simulink model "ModelCLLCController"  (R2026a)
settings: Solver=ode23t  StopTime=5e-3  FixedStep=1e-4  MaxStep=1e-6  AbsTol=1e-3
PreLoadFcn:
  | % Parameterize the model
  | 
  | if ~exist('CLLCDesign', 'var')
  | CLLCConverterDefaultInputParameters;
  | end
undefined symbols (not defined in the file or in its folder): CLLCController
libraries: fl_lib x46, nesl_utility x45, ee_lib x35, ConverterLibrary x1
(part 2 of 4)

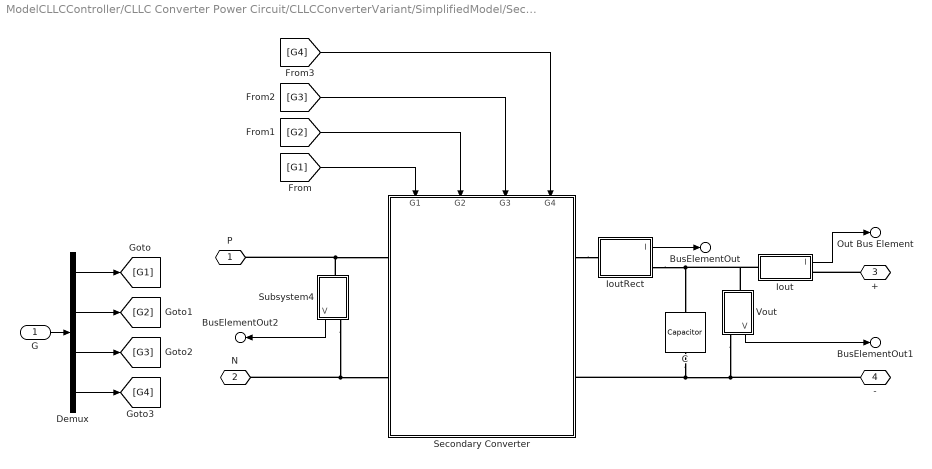
== system ModelCLLCController/CLLC Converter Power Circuit/CLLCConverterVariant/SimplifiedModel/Secondary Converter ==
  G : Inport
  C : fl_lib/Electrical/Electrical Elements/Capacitor  c=Co F  r=Rco Ohm  g=0 1/Ohm  i_specify=off  i_priority=None  i=0 A  i_nominal_specify=off  i_nominal_value=1  i_nominal_unit=A  v_specify=off  v_priority=None  v=450 V  v_nominal_specify=off  v_nominal_value=1  v_nominal_unit=V  vc_specify=on  vc_priority=High  vc=Vco V  vc_nominal_specify=off  vc_nominal_value=1  vc_nominal_unit=V
  Demux : Demux
  Iout : Subsystem
      mask Display: disp("I")
  IoutRect : Subsystem
      mask Display: disp("I")
  Secondary Converter : Subsystem  VariantControl=IdealSwitch
      settings: PortSchema="{\"entries\":[{\"content\":{\"sides\":[{\"content\":{\"connectorIds\":[\"LConn1\",\"LConn2\"]},\"type\":\"ConnectorPlacement.EquallySpacedRectSide\",\"uuid\":\"27c41940-d662-4779-afdd-48b642f77411\"},{\"content\":{\"connectorIds\":[\"RConn1\",\"RConn2\"],\"side\":\"RIGHT\"},\"type\":\"ConnectorPlacement.EquallySpacedRectSide\",\"uuid\":\"b0072b01-add1-4b0f-b94e-e1b6c9886b0e\"},{\"content\":{\"connectorIds\":[\"In1\",\"In2\",\"In3\",\"In4\"],\"side\":\"TOP\"},\"type\":\"ConnectorPlacement.EquallySpacedRectSide\",\"uuid\":\"c43bed80-422d-49db-9596-8b38d5c3e411\"},{\"content\":{\"side\":\"BOTTOM\"},\"type\":\"ConnectorPlacement.EquallySpacedRectSide\",\"uuid\":\"01f06046-f57e-45b0-bca5-368a5a543f97\"}]},\"type\":\"ConnectorPlacement.EquallySpacedConnector\",\"uuid\":\"2fcb5370-6bd7-4702-bf87-ebedbb7e376c\"}],\"packageUris\":[\"http://schema.mathworks.com/mf0/Connector/R2020b\"],\"version\":\"1.0\"}"
  Subsystem4 : Subsystem
      settings: PortSchema="{\"entries\":[{\"content\":{\"sides\":[{\"content\":{\"connectorIds\":[\"LConn1\"]},\"type\":\"ConnectorPlacement.EquallySpacedRectSide\",\"uuid\":\"e749c2ff-fd60-426f-a769-b61a7dfe80d2\"},{\"content\":{\"connectorIds\":[\"RConn1\",\"Out1\"],\"side\":\"RIGHT\"},\"type\":\"ConnectorPlacement.EquallySpacedRectSide\",\"uuid\":\"f3bb02bd-f8d2-4326-b68c-6f969fa4ac22\"},{\"content\":{\"side\":\"TOP\"},\"type\":\"ConnectorPlacement.EquallySpacedRectSide\",\"uuid\":\"9ab7a0d1-20d8-49e4-8eb3-54d34434204c\"}]},\"type\":\"ConnectorPlacement.EquallySpacedConnector\",\"uuid\":\"19e2a6d5-13f4-47de-bb59-b826817cba83\"}],\"packageUris\":[\"http://schema.mathworks.com/mf0/Connector/R2020b\"],\"version\":\"1.0\"}"
      mask Display: disp("V")
  Vout : Subsystem
      settings: PortSchema="{\"entries\":[{\"content\":{\"sides\":[{\"content\":{\"connectorIds\":[\"LConn1\"]},\"type\":\"ConnectorPlacement.EquallySpacedRectSide\",\"uuid\":\"e749c2ff-fd60-426f-a769-b61a7dfe80d2\"},{\"content\":{\"connectorIds\":[\"RConn1\",\"Out1\"],\"side\":\"RIGHT\"},\"type\":\"ConnectorPlacement.EquallySpacedRectSide\",\"uuid\":\"f3bb02bd-f8d2-4326-b68c-6f969fa4ac22\"},{\"content\":{\"side\":\"TOP\"},\"type\":\"ConnectorPlacement.EquallySpacedRectSide\",\"uuid\":\"9ab7a0d1-20d8-49e4-8eb3-54d34434204c\"}]},\"type\":\"ConnectorPlacement.EquallySpacedConnector\",\"uuid\":\"19e2a6d5-13f4-47de-bb59-b826817cba83\"}],\"packageUris\":[\"http://schema.mathworks.com/mf0/Connector/R2020b\"],\"version\":\"1.0\"}"
      mask Display: disp("V")
  P : PMIOPort  Side=Left
  N : PMIOPort  Port=2  Side=Left
  + : PMIOPort  Port=3  Side=Right
  - : PMIOPort  Port=4  Side=Right
  Out Bus Element : Outport  PortName=meas  Element=Iout [A]
  BusElementOut : Outport  PortName=meas  Element=IL [A]
  BusElementOut1 : Outport  PortName=meas  Element=Vout [V]
  BusElementOut2 : Outport  PortName=meas  Element=Vac [V]
  wires:
  Iout/1(I) -> Out Bus Element/1
  IoutRect/1(I) -> BusElementOut/1
  Vout/1(V) -> BusElementOut1/1
  Subsystem4/1(V) -> BusElementOut2/1
  Demux/2 -> [G2]
  Demux/1 -> [G1]
  G/1 -> Demux/1
  Demux/4 -> [G4]
  Demux/3 -> [G3]
  [G2] -> Secondary Converter/2(G2)
  [G3] -> Secondary Converter/3(G3)
  [G1] -> Secondary Converter/1(G1)
  [G4] -> Secondary Converter/4(G4)
  connections:
  Secondary Converter/RConn1 -- IoutRect/LConn1
  Subsystem4/RConn1 -- N/RConn1 -- Secondary Converter/LConn2
  Subsystem4/LConn1 -- P/RConn1 -- Secondary Converter/LConn1
  C/RConn1 -- -/RConn1 -- Vout/RConn1 -- Secondary Converter/RConn2
  IoutRect/RConn1 -- Iout/LConn1 -- Vout/LConn1 -- C/LConn1
  +/RConn1 -- Iout/RConn1

== system ModelCLLCController/CLLC Converter Power Circuit/CLLCConverterVariant/DetailedModel/Primary Converter/Iin ==
  Current Sensor : fl_lib/Electrical/Electrical Sensors/Current Sensor
  PS-Simulink Converter : nesl_utility/PS-Simulink Converter  PhysicalDomain=network_engine_domain  SubClassName=ps_output  LeftPortType=input  RightPortType=output  PseudoPeriodic=off  Frequencies=[]  VectorFormat=inherit  Unit=inherit  AffineConversion=off
  + : PMIOPort  Side=Left
  - : PMIOPort  Port=2  Side=Right
  I : Outport
  wires:
  PS-Simulink Converter/1 -> I/1
  connections:
  Current Sensor/RConn2 -- -/RConn1
  +/RConn1 -- Current Sensor/LConn1
  Current Sensor/RConn1 -- PS-Simulink Converter/LConn1

== system ModelCLLCController/CLLC Converter Power Circuit/CLLCConverterVariant/DetailedModel/Primary Converter/Primary Converter Full Bridge ==
  G1 : Inport
  G2 : Inport  Port=2
  G3 : Inport  Port=3
  G4 : Inport  Port=4
  Ideal MOSFET with Thermal : Subsystem  VariantControl=IdealMOSFETwithThermal
      settings: PortSchema="{\"entries\":[{\"content\":{\"sides\":[{\"content\":{\"connectorIds\":[\"LConn1\",\"LConn2\"]},\"type\":\"ConnectorPlacement.EquallySpacedRectSide\",\"uuid\":\"27c41940-d662-4779-afdd-48b642f77411\"},{\"content\":{\"connectorIds\":[\"RConn1\",\"RConn2\"],\"side\":\"RIGHT\"},\"type\":\"ConnectorPlacement.EquallySpacedRectSide\",\"uuid\":\"b0072b01-add1-4b0f-b94e-e1b6c9886b0e\"},{\"content\":{\"connectorIds\":[\"In1\",\"In2\",\"In3\",\"In4\"],\"side\":\"TOP\"},\"type\":\"ConnectorPlacement.EquallySpacedRectSide\",\"uuid\":\"c43bed80-422d-49db-9596-8b38d5c3e411\"},{\"content\":{\"side\":\"BOTTOM\"},\"type\":\"ConnectorPlacement.EquallySpacedRectSide\",\"uuid\":\"01f06046-f57e-45b0-bca5-368a5a543f97\"}]},\"type\":\"ConnectorPlacement.EquallySpacedConnector\",\"uuid\":\"2fcb5370-6bd7-4702-bf87-ebedbb7e376c\"}],\"packageUris\":[\"http://schema.mathworks.com/mf0/Connector/R2020b\"],\"version\":\"1.0\"}"
  Ideal Switch : Subsystem  VariantControl=IdealSwitch
      settings: PortSchema="{\"entries\":[{\"content\":{\"sides\":[{\"content\":{\"connectorIds\":[\"LConn1\",\"LConn2\"]},\"type\":\"ConnectorPlacement.EquallySpacedRectSide\",\"uuid\":\"27c41940-d662-4779-afdd-48b642f77411\"},{\"content\":{\"connectorIds\":[\"RConn1\",\"RConn2\"],\"side\":\"RIGHT\"},\"type\":\"ConnectorPlacement.EquallySpacedRectSide\",\"uuid\":\"b0072b01-add1-4b0f-b94e-e1b6c9886b0e\"},{\"content\":{\"connectorIds\":[\"In1\",\"In2\",\"In3\",\"In4\"],\"side\":\"TOP\"},\"type\":\"ConnectorPlacement.EquallySpacedRectSide\",\"uuid\":\"c43bed80-422d-49db-9596-8b38d5c3e411\"},{\"content\":{\"side\":\"BOTTOM\"},\"type\":\"ConnectorPlacement.EquallySpacedRectSide\",\"uuid\":\"01f06046-f57e-45b0-bca5-368a5a543f97\"}]},\"type\":\"ConnectorPlacement.EquallySpacedConnector\",\"uuid\":\"2fcb5370-6bd7-4702-bf87-ebedbb7e376c\"}],\"packageUris\":[\"http://schema.mathworks.com/mf0/Connector/R2020b\"],\"version\":\"1.0\"}"
  P1 : PMIOPort  Side=Left
  N1 : PMIOPort  Port=2  Side=Left
  P2 : PMIOPort  Port=3  Side=Right
  N2 : PMIOPort  Port=4  Side=Right

== system ModelCLLCController/CLLC Converter Power Circuit/CLLCConverterVariant/DetailedModel/Primary Converter/Vin ==
  PS-Simulink Converter : nesl_utility/PS-Simulink Converter  PhysicalDomain=network_engine_domain  SubClassName=ps_output  LeftPortType=input  RightPortType=output  PseudoPeriodic=off  Frequencies=[]  VectorFormat=inherit  Unit=inherit  AffineConversion=off
  Voltage Sensor : fl_lib/Electrical/Electrical Sensors/Voltage Sensor
  + : PMIOPort  Side=Left
  - : PMIOPort  Port=2  Side=Right
  V : Outport
  wires:
  PS-Simulink Converter/1 -> V/1
  connections:
  Voltage Sensor/RConn2 -- -/RConn1
  Voltage Sensor/LConn1 -- +/RConn1
  PS-Simulink Converter/LConn1 -- Voltage Sensor/RConn1

== system ModelCLLCController/CLLC Converter Power Circuit/CLLCConverterVariant/DetailedModel/Resonant Tank/Ip ==
  Current Sensor : fl_lib/Electrical/Electrical Sensors/Current Sensor
  PS-Simulink Converter : nesl_utility/PS-Simulink Converter  PhysicalDomain=network_engine_domain  SubClassName=ps_output  LeftPortType=input  RightPortType=output  PseudoPeriodic=off  Frequencies=[]  VectorFormat=inherit  Unit=inherit  AffineConversion=off
  + : PMIOPort  Side=Left
  - : PMIOPort  Port=2  Side=Right
  I : Outport
  wires:
  PS-Simulink Converter/1 -> I/1
  connections:
  Current Sensor/RConn2 -- -/RConn1
  +/RConn1 -- Current Sensor/LConn1
  Current Sensor/RConn1 -- PS-Simulink Converter/LConn1

== system ModelCLLCController/CLLC Converter Power Circuit/CLLCConverterVariant/DetailedModel/Resonant Tank/Is ==
  Current Sensor : fl_lib/Electrical/Electrical Sensors/Current Sensor
  PS-Simulink Converter : nesl_utility/PS-Simulink Converter  PhysicalDomain=network_engine_domain  SubClassName=ps_output  LeftPortType=input  RightPortType=output  PseudoPeriodic=off  Frequencies=[]  VectorFormat=inherit  Unit=inherit  AffineConversion=off
  + : PMIOPort  Side=Left
  - : PMIOPort  Port=2  Side=Right
  I : Outport
  wires:
  PS-Simulink Converter/1 -> I/1
  connections:
  Current Sensor/RConn2 -- -/RConn1
  +/RConn1 -- Current Sensor/LConn1
  Current Sensor/RConn1 -- PS-Simulink Converter/LConn1

== system ModelCLLCController/CLLC Converter Power Circuit/CLLCConverterVariant/DetailedModel/Resonant Tank/Vp ==
  PS-Simulink Converter : nesl_utility/PS-Simulink Converter  PhysicalDomain=network_engine_domain  SubClassName=ps_output  LeftPortType=input  RightPortType=output  PseudoPeriodic=off  Frequencies=[]  VectorFormat=inherit  Unit=inherit  AffineConversion=off
  Voltage Sensor : fl_lib/Electrical/Electrical Sensors/Voltage Sensor
  + : PMIOPort  Side=Left
  - : PMIOPort  Port=2  Side=Right
  V : Outport
  wires:
  PS-Simulink Converter/1 -> V/1
  connections:
  Voltage Sensor/RConn2 -- -/RConn1
  Voltage Sensor/LConn1 -- +/RConn1
  PS-Simulink Converter/LConn1 -- Voltage Sensor/RConn1

== system ModelCLLCController/CLLC Converter Power Circuit/CLLCConverterVariant/DetailedModel/Resonant Tank/Vs ==
  PS-Simulink Converter : nesl_utility/PS-Simulink Converter  PhysicalDomain=network_engine_domain  SubClassName=ps_output  LeftPortType=input  RightPortType=output  PseudoPeriodic=off  Frequencies=[]  VectorFormat=inherit  Unit=inherit  AffineConversion=off
  Voltage Sensor : fl_lib/Electrical/Electrical Sensors/Voltage Sensor
  + : PMIOPort  Side=Left
  - : PMIOPort  Port=2  Side=Right
  V : Outport
  wires:
  PS-Simulink Converter/1 -> V/1
  connections:
  Voltage Sensor/RConn2 -- -/RConn1
  Voltage Sensor/LConn1 -- +/RConn1
  PS-Simulink Converter/LConn1 -- Voltage Sensor/RConn1

== system ModelCLLCController/CLLC Converter Power Circuit/CLLCConverterVariant/DetailedModel/Secondary Converter/Iout ==
  Current Sensor : fl_lib/Electrical/Electrical Sensors/Current Sensor
  PS-Simulink Converter : nesl_utility/PS-Simulink Converter  PhysicalDomain=network_engine_domain  SubClassName=ps_output  LeftPortType=input  RightPortType=output  PseudoPeriodic=off  Frequencies=[]  VectorFormat=inherit  Unit=inherit  AffineConversion=off
  + : PMIOPort  Side=Left
  - : PMIOPort  Port=2  Side=Right
  I : Outport
  wires:
  PS-Simulink Converter/1 -> I/1
  connections:
  Current Sensor/RConn2 -- -/RConn1
  +/RConn1 -- Current Sensor/LConn1
  Current Sensor/RConn1 -- PS-Simulink Converter/LConn1

== system ModelCLLCController/CLLC Converter Power Circuit/CLLCConverterVariant/DetailedModel/Secondary Converter/IoutRect ==
  Current Sensor : fl_lib/Electrical/Electrical Sensors/Current Sensor
  PS-Simulink Converter : nesl_utility/PS-Simulink Converter  PhysicalDomain=network_engine_domain  SubClassName=ps_output  LeftPortType=input  RightPortType=output  PseudoPeriodic=off  Frequencies=[]  VectorFormat=inherit  Unit=inherit  AffineConversion=off
  + : PMIOPort  Side=Left
  - : PMIOPort  Port=2  Side=Right
  I : Outport
  wires:
  PS-Simulink Converter/1 -> I/1
  connections:
  Current Sensor/RConn2 -- -/RConn1
  +/RConn1 -- Current Sensor/LConn1
  Current Sensor/RConn1 -- PS-Simulink Converter/LConn1

== system ModelCLLCController/CLLC Converter Power Circuit/CLLCConverterVariant/DetailedModel/Secondary Converter/Secondary Converter Full Bridge ==
  G1 : Inport
  G2 : Inport  Port=2
  G3 : Inport  Port=3
  G4 : Inport  Port=4
  Ideal MOSFET with Thermal : Subsystem  VariantControl=IdealMOSFETwithThermal
      settings: PortSchema="{\"entries\":[{\"content\":{\"sides\":[{\"content\":{\"connectorIds\":[\"LConn1\",\"LConn2\"]},\"type\":\"ConnectorPlacement.EquallySpacedRectSide\",\"uuid\":\"27c41940-d662-4779-afdd-48b642f77411\"},{\"content\":{\"connectorIds\":[\"RConn1\",\"RConn2\"],\"side\":\"RIGHT\"},\"type\":\"ConnectorPlacement.EquallySpacedRectSide\",\"uuid\":\"b0072b01-add1-4b0f-b94e-e1b6c9886b0e\"},{\"content\":{\"connectorIds\":[\"In1\",\"In2\",\"In3\",\"In4\"],\"side\":\"TOP\"},\"type\":\"ConnectorPlacement.EquallySpacedRectSide\",\"uuid\":\"c43bed80-422d-49db-9596-8b38d5c3e411\"},{\"content\":{\"side\":\"BOTTOM\"},\"type\":\"ConnectorPlacement.EquallySpacedRectSide\",\"uuid\":\"01f06046-f57e-45b0-bca5-368a5a543f97\"}]},\"type\":\"ConnectorPlacement.EquallySpacedConnector\",\"uuid\":\"2fcb5370-6bd7-4702-bf87-ebedbb7e376c\"}],\"packageUris\":[\"http://schema.mathworks.com/mf0/Connector/R2020b\"],\"version\":\"1.0\"}"
  Ideal Switch : Subsystem  VariantControl=IdealSwitch
      settings: PortSchema="{\"entries\":[{\"content\":{\"sides\":[{\"content\":{\"connectorIds\":[\"LConn1\",\"LConn2\"]},\"type\":\"ConnectorPlacement.EquallySpacedRectSide\",\"uuid\":\"27c41940-d662-4779-afdd-48b642f77411\"},{\"content\":{\"connectorIds\":[\"RConn1\",\"RConn2\"],\"side\":\"RIGHT\"},\"type\":\"ConnectorPlacement.EquallySpacedRectSide\",\"uuid\":\"b0072b01-add1-4b0f-b94e-e1b6c9886b0e\"},{\"content\":{\"connectorIds\":[\"In1\",\"In2\",\"In3\",\"In4\"],\"side\":\"TOP\"},\"type\":\"ConnectorPlacement.EquallySpacedRectSide\",\"uuid\":\"c43bed80-422d-49db-9596-8b38d5c3e411\"},{\"content\":{\"side\":\"BOTTOM\"},\"type\":\"ConnectorPlacement.EquallySpacedRectSide\",\"uuid\":\"01f06046-f57e-45b0-bca5-368a5a543f97\"}]},\"type\":\"ConnectorPlacement.EquallySpacedConnector\",\"uuid\":\"2fcb5370-6bd7-4702-bf87-ebedbb7e376c\"}],\"packageUris\":[\"http://schema.mathworks.com/mf0/Connector/R2020b\"],\"version\":\"1.0\"}"
  P1 : PMIOPort  Side=Right
  N1 : PMIOPort  Port=2  Side=Right
  P2 : PMIOPort  Port=3  Side=Left
  N2 : PMIOPort  Port=4  Side=Left

== system ModelCLLCController/CLLC Converter Power Circuit/CLLCConverterVariant/DetailedModel/Secondary Converter/Subsystem4 ==
  PS-Simulink Converter : nesl_utility/PS-Simulink Converter  PhysicalDomain=network_engine_domain  SubClassName=ps_output  LeftPortType=input  RightPortType=output  PseudoPeriodic=off  Frequencies=[]  VectorFormat=inherit  Unit=inherit  AffineConversion=off
  Voltage Sensor : fl_lib/Electrical/Electrical Sensors/Voltage Sensor
  + : PMIOPort  Side=Left
  - : PMIOPort  Port=2  Side=Right
  V : Outport
  wires:
  PS-Simulink Converter/1 -> V/1
  connections:
  Voltage Sensor/RConn2 -- -/RConn1
  Voltage Sensor/LConn1 -- +/RConn1
  PS-Simulink Converter/LConn1 -- Voltage Sensor/RConn1

== system ModelCLLCController/CLLC Converter Power Circuit/CLLCConverterVariant/DetailedModel/Secondary Converter/Vout ==
  PS-Simulink Converter : nesl_utility/PS-Simulink Converter  PhysicalDomain=network_engine_domain  SubClassName=ps_output  LeftPortType=input  RightPortType=output  PseudoPeriodic=off  Frequencies=[]  VectorFormat=inherit  Unit=inherit  AffineConversion=off
  Voltage Sensor : fl_lib/Electrical/Electrical Sensors/Voltage Sensor
  + : PMIOPort  Side=Left
  - : PMIOPort  Port=2  Side=Right
  V : Outport
  wires:
  PS-Simulink Converter/1 -> V/1
  connections:
  Voltage Sensor/RConn2 -- -/RConn1
  Voltage Sensor/LConn1 -- +/RConn1
  PS-Simulink Converter/LConn1 -- Voltage Sensor/RConn1

== system ModelCLLCController/CLLC Converter Power Circuit/CLLCConverterVariant/SimplifiedModel/Primary Converter/Iin ==
  Current Sensor : fl_lib/Electrical/Electrical Sensors/Current Sensor
  PS-Simulink Converter : nesl_utility/PS-Simulink Converter  PhysicalDomain=network_engine_domain  SubClassName=ps_output  LeftPortType=input  RightPortType=output  PseudoPeriodic=off  Frequencies=[]  VectorFormat=inherit  Unit=inherit  AffineConversion=off
  + : PMIOPort  Side=Left
  - : PMIOPort  Port=2  Side=Right
  I : Outport
  wires:
  PS-Simulink Converter/1 -> I/1
  connections:
  Current Sensor/RConn1 -- PS-Simulink Converter/LConn1
  +/RConn1 -- Current Sensor/LConn1
  Current Sensor/RConn2 -- -/RConn1

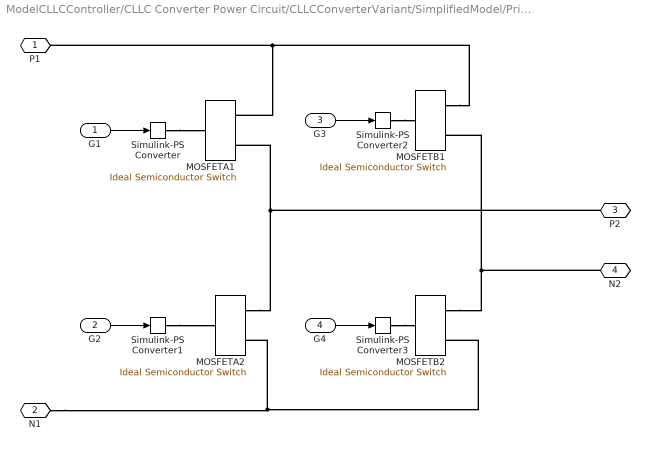
== system ModelCLLCController/CLLC Converter Power Circuit/CLLCConverterVariant/SimplifiedModel/Primary Converter/Primary Converter ==
  G1 : Inport
  G2 : Inport  Port=2
  G3 : Inport  Port=3
  G4 : Inport  Port=4
  MOSFETA1 : ee_lib/Semiconductors & Converters/Ideal Semiconductor Switch  port_option=ee.enum.controlport.ps  Ron=PrimaryRon Ohm  Goff=PrimaryGoff 1/Ohm  Vth=PrimaryVth V  diode_param=ee.enum.semiconductors.protectionDiode.nodynamics  diode_Vf=PrimaryVbodydiodeOn V  diode_Ron=PrimaryRbodydiodeOn Ohm  diode_Goff=PrimaryGbodydiodeOff 1/Ohm  diode_C=50e-9 F  diode_iRM=-235 A  diode_iF=300 A  diode_idot=-50 A/us  diode_trr_param=ee.enum.converters.diodetrr.trr_factor  diode_trr_factor=3  diode_trr=15 us  diode_Qrr=1500 s*uA
  MOSFETA2 : ee_lib/Semiconductors & Converters/Ideal Semiconductor Switch  port_option=ee.enum.controlport.ps  Ron=PrimaryRon Ohm  Goff=PrimaryGoff 1/Ohm  Vth=PrimaryVth V  diode_param=ee.enum.semiconductors.protectionDiode.nodynamics  diode_Vf=PrimaryVbodydiodeOn V  diode_Ron=PrimaryRbodydiodeOn Ohm  diode_Goff=PrimaryGbodydiodeOff 1/Ohm  diode_C=50e-9 F  diode_iRM=-235 A  diode_iF=300 A  diode_idot=-50 A/us  diode_trr_param=ee.enum.converters.diodetrr.trr_factor  diode_trr_factor=3  diode_trr=15 us  diode_Qrr=1500 s*uA
  MOSFETB1 : ee_lib/Semiconductors & Converters/Ideal Semiconductor Switch  port_option=ee.enum.controlport.ps  Ron=PrimaryRon Ohm  Goff=PrimaryGoff 1/Ohm  Vth=PrimaryVth V  diode_param=ee.enum.semiconductors.protectionDiode.nodynamics  diode_Vf=PrimaryVbodydiodeOn V  diode_Ron=PrimaryRbodydiodeOn Ohm  diode_Goff=PrimaryGbodydiodeOff 1/Ohm  diode_C=50e-9 F  diode_iRM=-235 A  diode_iF=300 A  diode_idot=-50 A/us  diode_trr_param=ee.enum.converters.diodetrr.trr_factor  diode_trr_factor=3  diode_trr=15 us  diode_Qrr=1500 s*uA
  MOSFETB2 : ee_lib/Semiconductors & Converters/Ideal Semiconductor Switch  port_option=ee.enum.controlport.ps  Ron=PrimaryRon Ohm  Goff=PrimaryGoff 1/Ohm  Vth=PrimaryVth V  diode_param=ee.enum.semiconductors.protectionDiode.nodynamics  diode_Vf=PrimaryVbodydiodeOn V  diode_Ron=PrimaryRbodydiodeOn Ohm  diode_Goff=PrimaryGbodydiodeOff 1/Ohm  diode_C=50e-9 F  diode_iRM=-235 A  diode_iF=300 A  diode_idot=-50 A/us  diode_trr_param=ee.enum.converters.diodetrr.trr_factor  diode_trr_factor=3  diode_trr=15 us  diode_Qrr=1500 s*uA
  Simulink-PS Converter{,1..3} (4 alike) : nesl_utility/Simulink-PS Converter  PhysicalDomain=network_engine_domain  SubClassName=ps_input  LeftPortType=input  RightPortType=output  PseudoPeriodic=off  Frequencies=[]  NoiseDistribution=none  NoiseParameters=[]  Unit=1  AffineConversion=off  FilteringAndDerivatives=provide  SimscapeFilterOrder=1  InputFilterTimeConstant=0.001  UdotUserProvided=0
  P1 : PMIOPort  Side=Left
  N1 : PMIOPort  Port=2  Side=Left
  P2 : PMIOPort  Port=3  Side=Right
  N2 : PMIOPort  Port=4  Side=Right
  wires:
  G4/1 -> Simulink-PS Converter3/1
  G3/1 -> Simulink-PS Converter2/1
  G2/1 -> Simulink-PS Converter1/1
  G1/1 -> Simulink-PS Converter/1
  connections:
  Simulink-PS Converter3/RConn1 -- MOSFETB2/LConn1
  Simulink-PS Converter2/RConn1 -- MOSFETB1/LConn1
  Simulink-PS Converter1/RConn1 -- MOSFETA2/LConn1
  Simulink-PS Converter/RConn1 -- MOSFETA1/LConn1
  MOSFETA2/RConn2 -- MOSFETB2/RConn2 -- N1/RConn1
  MOSFETA1/RConn1 -- MOSFETB1/RConn1 -- P1/RConn1
  MOSFETA1/RConn2 -- MOSFETA2/RConn1 -- P2/RConn1
  MOSFETB1/RConn2 -- MOSFETB2/RConn1 -- N2/RConn1

== system ModelCLLCController/CLLC Converter Power Circuit/CLLCConverterVariant/SimplifiedModel/Primary Converter/Vin ==
  PS-Simulink Converter : nesl_utility/PS-Simulink Converter  PhysicalDomain=network_engine_domain  SubClassName=ps_output  LeftPortType=input  RightPortType=output  PseudoPeriodic=off  Frequencies=[]  VectorFormat=inherit  Unit=inherit  AffineConversion=off
  Voltage Sensor : fl_lib/Electrical/Electrical Sensors/Voltage Sensor
  + : PMIOPort  Side=Left
  - : PMIOPort  Port=2  Side=Right
  V : Outport
  wires:
  PS-Simulink Converter/1 -> V/1
  connections:
  PS-Simulink Converter/LConn1 -- Voltage Sensor/RConn1
  Voltage Sensor/LConn1 -- +/RConn1
  Voltage Sensor/RConn2 -- -/RConn1

== system ModelCLLCController/CLLC Converter Power Circuit/CLLCConverterVariant/SimplifiedModel/Resonant Tank/Ip ==
  Current Sensor : fl_lib/Electrical/Electrical Sensors/Current Sensor
  PS-Simulink Converter : nesl_utility/PS-Simulink Converter  PhysicalDomain=network_engine_domain  SubClassName=ps_output  LeftPortType=input  RightPortType=output  PseudoPeriodic=off  Frequencies=[]  VectorFormat=inherit  Unit=inherit  AffineConversion=off
  + : PMIOPort  Side=Left
  - : PMIOPort  Port=2  Side=Right
  I : Outport
  wires:
  PS-Simulink Converter/1 -> I/1
  connections:
  Current Sensor/RConn1 -- PS-Simulink Converter/LConn1
  +/RConn1 -- Current Sensor/LConn1
  Current Sensor/RConn2 -- -/RConn1

== system ModelCLLCController/CLLC Converter Power Circuit/CLLCConverterVariant/SimplifiedModel/Resonant Tank/Is ==
  Current Sensor : fl_lib/Electrical/Electrical Sensors/Current Sensor
  PS-Simulink Converter : nesl_utility/PS-Simulink Converter  PhysicalDomain=network_engine_domain  SubClassName=ps_output  LeftPortType=input  RightPortType=output  PseudoPeriodic=off  Frequencies=[]  VectorFormat=inherit  Unit=inherit  AffineConversion=off
  + : PMIOPort  Side=Left
  - : PMIOPort  Port=2  Side=Right
  I : Outport
  wires:
  PS-Simulink Converter/1 -> I/1
  connections:
  Current Sensor/RConn1 -- PS-Simulink Converter/LConn1
  +/RConn1 -- Current Sensor/LConn1
  Current Sensor/RConn2 -- -/RConn1

== system ModelCLLCController/CLLC Converter Power Circuit/CLLCConverterVariant/SimplifiedModel/Resonant Tank/Vp ==
  PS-Simulink Converter : nesl_utility/PS-Simulink Converter  PhysicalDomain=network_engine_domain  SubClassName=ps_output  LeftPortType=input  RightPortType=output  PseudoPeriodic=off  Frequencies=[]  VectorFormat=inherit  Unit=inherit  AffineConversion=off
  Voltage Sensor : fl_lib/Electrical/Electrical Sensors/Voltage Sensor
  + : PMIOPort  Side=Left
  - : PMIOPort  Port=2  Side=Right
  V : Outport
  wires:
  PS-Simulink Converter/1 -> V/1
  connections:
  PS-Simulink Converter/LConn1 -- Voltage Sensor/RConn1
  Voltage Sensor/LConn1 -- +/RConn1
  Voltage Sensor/RConn2 -- -/RConn1

== system ModelCLLCController/CLLC Converter Power Circuit/CLLCConverterVariant/SimplifiedModel/Resonant Tank/Vs ==
  PS-Simulink Converter : nesl_utility/PS-Simulink Converter  PhysicalDomain=network_engine_domain  SubClassName=ps_output  LeftPortType=input  RightPortType=output  PseudoPeriodic=off  Frequencies=[]  VectorFormat=inherit  Unit=inherit  AffineConversion=off
  Voltage Sensor : fl_lib/Electrical/Electrical Sensors/Voltage Sensor
  + : PMIOPort  Side=Left
  - : PMIOPort  Port=2  Side=Right
  V : Outport
  wires:
  PS-Simulink Converter/1 -> V/1
  connections:
  PS-Simulink Converter/LConn1 -- Voltage Sensor/RConn1
  Voltage Sensor/LConn1 -- +/RConn1
  Voltage Sensor/RConn2 -- -/RConn1

== system ModelCLLCController/CLLC Converter Power Circuit/CLLCConverterVariant/SimplifiedModel/Secondary Converter/Iout ==
  Current Sensor : fl_lib/Electrical/Electrical Sensors/Current Sensor
  PS-Simulink Converter : nesl_utility/PS-Simulink Converter  PhysicalDomain=network_engine_domain  SubClassName=ps_output  LeftPortType=input  RightPortType=output  PseudoPeriodic=off  Frequencies=[]  VectorFormat=inherit  Unit=inherit  AffineConversion=off
  + : PMIOPort  Side=Left
  - : PMIOPort  Port=2  Side=Right
  I : Outport
  wires:
  PS-Simulink Converter/1 -> I/1
  connections:
  Current Sensor/RConn1 -- PS-Simulink Converter/LConn1
  +/RConn1 -- Current Sensor/LConn1
  Current Sensor/RConn2 -- -/RConn1

== system ModelCLLCController/CLLC Converter Power Circuit/CLLCConverterVariant/SimplifiedModel/Secondary Converter/IoutRect ==
  Current Sensor : fl_lib/Electrical/Electrical Sensors/Current Sensor
  PS-Simulink Converter : nesl_utility/PS-Simulink Converter  PhysicalDomain=network_engine_domain  SubClassName=ps_output  LeftPortType=input  RightPortType=output  PseudoPeriodic=off  Frequencies=[]  VectorFormat=inherit  Unit=inherit  AffineConversion=off
  + : PMIOPort  Side=Left
  - : PMIOPort  Port=2  Side=Right
  I : Outport
  wires:
  PS-Simulink Converter/1 -> I/1
  connections:
  Current Sensor/RConn1 -- PS-Simulink Converter/LConn1
  +/RConn1 -- Current Sensor/LConn1
  Current Sensor/RConn2 -- -/RConn1

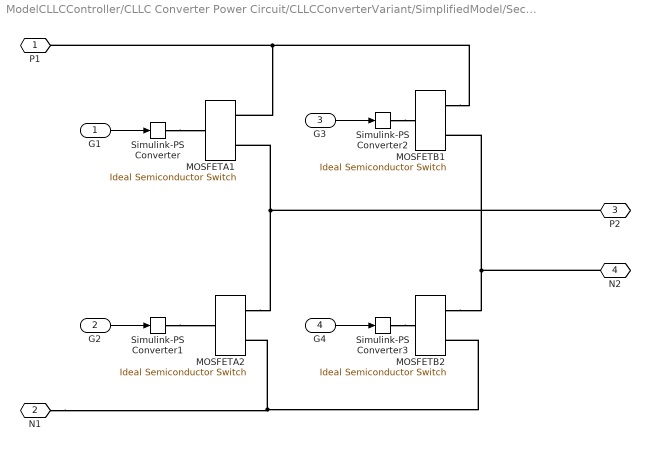
== system ModelCLLCController/CLLC Converter Power Circuit/CLLCConverterVariant/SimplifiedModel/Secondary Converter/Secondary Converter ==
  G1 : Inport
  G2 : Inport  Port=2
  G3 : Inport  Port=3
  G4 : Inport  Port=4
  MOSFETA1 : ee_lib/Semiconductors & Converters/Ideal Semiconductor Switch  port_option=ee.enum.controlport.ps  Ron=SecondaryRon Ohm  Goff=SecondaryGoff 1/Ohm  Vth=SecondaryVth V  diode_param=ee.enum.semiconductors.protectionDiode.nodynamics  diode_Vf=SecondaryVbodydiodeOn V  diode_Ron=SecondaryRbodydiodeOn Ohm  diode_Goff=SecondaryGbodydiodeOff 1/Ohm  diode_C=50e-9 F  diode_iRM=-235 A  diode_iF=300 A  diode_idot=-50 A/us  diode_trr_param=ee.enum.converters.diodetrr.trr_factor  diode_trr_factor=3  diode_trr=15 us  diode_Qrr=1500 s*uA
  MOSFETA2 : ee_lib/Semiconductors & Converters/Ideal Semiconductor Switch  port_option=ee.enum.controlport.ps  Ron=SecondaryRon Ohm  Goff=SecondaryGoff 1/Ohm  Vth=SecondaryVth V  diode_param=ee.enum.semiconductors.protectionDiode.nodynamics  diode_Vf=SecondaryVbodydiodeOn V  diode_Ron=SecondaryRbodydiodeOn Ohm  diode_Goff=SecondaryGbodydiodeOff 1/Ohm  diode_C=50e-9 F  diode_iRM=-235 A  diode_iF=300 A  diode_idot=-50 A/us  diode_trr_param=ee.enum.converters.diodetrr.trr_factor  diode_trr_factor=3  diode_trr=15 us  diode_Qrr=1500 s*uA
  MOSFETB1 : ee_lib/Semiconductors & Converters/Ideal Semiconductor Switch  port_option=ee.enum.controlport.ps  Ron=SecondaryRon Ohm  Goff=SecondaryGoff 1/Ohm  Vth=SecondaryVth V  diode_param=ee.enum.semiconductors.protectionDiode.nodynamics  diode_Vf=SecondaryVbodydiodeOn V  diode_Ron=SecondaryRbodydiodeOn Ohm  diode_Goff=SecondaryGbodydiodeOff 1/Ohm  diode_C=50e-9 F  diode_iRM=-235 A  diode_iF=300 A  diode_idot=-50 A/us  diode_trr_param=ee.enum.converters.diodetrr.trr_factor  diode_trr_factor=3  diode_trr=15 us  diode_Qrr=1500 s*uA
  MOSFETB2 : ee_lib/Semiconductors & Converters/Ideal Semiconductor Switch  port_option=ee.enum.controlport.ps  Ron=SecondaryRon Ohm  Goff=SecondaryGoff 1/Ohm  Vth=SecondaryVth V  diode_param=ee.enum.semiconductors.protectionDiode.nodynamics  diode_Vf=SecondaryVbodydiodeOn V  diode_Ron=SecondaryRbodydiodeOn Ohm  diode_Goff=SecondaryGbodydiodeOff 1/Ohm  diode_C=50e-9 F  diode_iRM=-235 A  diode_iF=300 A  diode_idot=-50 A/us  diode_trr_param=ee.enum.converters.diodetrr.trr_factor  diode_trr_factor=3  diode_trr=15 us  diode_Qrr=1500 s*uA
  Simulink-PS Converter{,1..3} (4 alike) : nesl_utility/Simulink-PS Converter  PhysicalDomain=network_engine_domain  SubClassName=ps_input  LeftPortType=input  RightPortType=output  PseudoPeriodic=off  Frequencies=[]  NoiseDistribution=none  NoiseParameters=[]  Unit=1  AffineConversion=off  FilteringAndDerivatives=provide  SimscapeFilterOrder=1  InputFilterTimeConstant=0.001  UdotUserProvided=0
  P1 : PMIOPort  Side=Right
  N1 : PMIOPort  Port=2  Side=Right
  P2 : PMIOPort  Port=3  Side=Left
  N2 : PMIOPort  Port=4  Side=Left
  wires:
  G4/1 -> Simulink-PS Converter3/1
  G3/1 -> Simulink-PS Converter2/1
  G2/1 -> Simulink-PS Converter1/1
  G1/1 -> Simulink-PS Converter/1
  connections:
  Simulink-PS Converter3/RConn1 -- MOSFETB2/LConn1
  Simulink-PS Converter2/RConn1 -- MOSFETB1/LConn1
  Simulink-PS Converter1/RConn1 -- MOSFETA2/LConn1
  Simulink-PS Converter/RConn1 -- MOSFETA1/LConn1
  MOSFETA2/RConn2 -- MOSFETB2/RConn2 -- N1/RConn1
  MOSFETA1/RConn1 -- MOSFETB1/RConn1 -- P1/RConn1
  MOSFETA1/RConn2 -- MOSFETA2/RConn1 -- P2/RConn1
  MOSFETB1/RConn2 -- MOSFETB2/RConn1 -- N2/RConn1

== system ModelCLLCController/CLLC Converter Power Circuit/CLLCConverterVariant/SimplifiedModel/Secondary Converter/Subsystem4 ==
  PS-Simulink Converter : nesl_utility/PS-Simulink Converter  PhysicalDomain=network_engine_domain  SubClassName=ps_output  LeftPortType=input  RightPortType=output  PseudoPeriodic=off  Frequencies=[]  VectorFormat=inherit  Unit=inherit  AffineConversion=off
  Voltage Sensor : fl_lib/Electrical/Electrical Sensors/Voltage Sensor
  + : PMIOPort  Side=Left
  - : PMIOPort  Port=2  Side=Right
  V : Outport
  wires:
  PS-Simulink Converter/1 -> V/1
  connections:
  PS-Simulink Converter/LConn1 -- Voltage Sensor/RConn1
  Voltage Sensor/LConn1 -- +/RConn1
  Voltage Sensor/RConn2 -- -/RConn1

== system ModelCLLCController/CLLC Converter Power Circuit/CLLCConverterVariant/SimplifiedModel/Secondary Converter/Vout ==
  PS-Simulink Converter : nesl_utility/PS-Simulink Converter  PhysicalDomain=network_engine_domain  SubClassName=ps_output  LeftPortType=input  RightPortType=output  PseudoPeriodic=off  Frequencies=[]  VectorFormat=inherit  Unit=inherit  AffineConversion=off
  Voltage Sensor : fl_lib/Electrical/Electrical Sensors/Voltage Sensor
  + : PMIOPort  Side=Left
  - : PMIOPort  Port=2  Side=Right
  V : Outport
  wires:
  PS-Simulink Converter/1 -> V/1
  connections:
  PS-Simulink Converter/LConn1 -- Voltage Sensor/RConn1
  Voltage Sensor/LConn1 -- +/RConn1
  Voltage Sensor/RConn2 -- -/RConn1
